simulink model "Intelligent_Microgrid_EMS"  (R2026b)
settings: Solver=FixedStepDiscrete  StopTime=24  FixedStep=1
undefined symbols (not defined in the file or in its folder): DiscIntNeverNeededParam
settings Model: Creator=Areeha  LastModifiedBy=Areeha

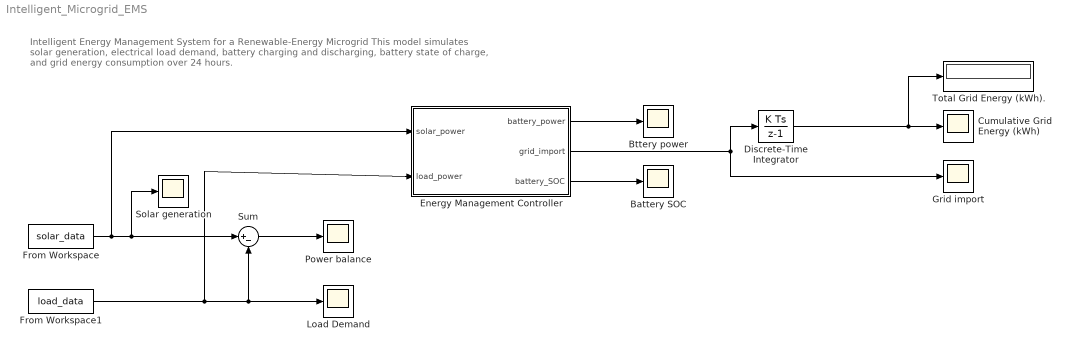
== system Intelligent_Microgrid_EMS ==
  note: Intelligent Energy Management System for a Renewable-Energy Microgrid This model simulates solar generation, electrical load demand, battery charging and discharging, battery state of charge, and grid energy consumption over 24 hours.
  Battery SOC : Scope
      settings: ActiveDisplayYMinimum=10.000000000000004  ActiveDisplayYMaximum=110  DataLoggingVariableName=ScopeData3
  Bttery power : Scope
      settings: ActiveDisplayYMinimum=-2.275  ActiveDisplayYMaximum=2.475
  Cumulative Grid Energy (kWh) : Scope
      settings: ActiveDisplayYMinimum=-2.2249999999999996  ActiveDisplayYMaximum=20.025000000000002  DataLoggingVariableName=ScopeData6
  Discrete-Time Integrator : DiscreteIntegrator  ICPrevOutput=DiscIntNeverNeededParam  ICPrevScaledInput=DiscIntNeverNeededParam
  Energy Management Controller : MATLAB Function  TreatAsAtomicUnit=on
  From Workspace : FromWorkspace  VariableName=solar_data
  From Workspace1 : FromWorkspace  VariableName=load_data
  Grid import : Scope
      settings: ActiveDisplayYMinimum=-0.37499999999999989  ActiveDisplayYMaximum=3.375  DataLoggingVariableName=ScopeData2
  Load Demand : Scope
      settings: ActiveDisplayYMinimum=0.40000000000000013  ActiveDisplayYMaximum=4.4  DataLoggingVariableName=ScopeData5
  Power balance : Scope
      settings: ActiveDisplayYMinimum=-4.725  ActiveDisplayYMaximum=2.525
  Solar generation : Scope
      settings: ActiveDisplayYMinimum=-0.62499999999999989  ActiveDisplayYMaximum=5.625  DataLoggingVariableName=ScopeData4
  Sum : Sum  Inputs=|+-
  Total Grid Energy (kWh). : Display
  wires:
  From Workspace/1 -> Energy Management Controller/1(solar_power), Solar generation/1, Sum/1
  From Workspace1/1 -> Load Demand/1, Sum/2, Energy Management Controller/2(load_power)
  Sum/1 -> Power balance/1
  Energy Management Controller/1(battery_power) -> Bttery power/1
  Energy Management Controller/2(grid_import) -> Grid import/1, Discrete-Time Integrator/1
  Energy Management Controller/3(battery_SOC) -> Battery SOC/1
  Discrete-Time Integrator/1 -> Total Grid Energy (kWh)./1, Cumulative Grid Energy (kWh)/1

== matlab function Intelligent_Microgrid_EMS/Energy Management Controller ==
  data: solar_power input; battery_power output; load_power input; grid_import output; battery_SOC output

function [battery_power, grid_import, battery_SOC] = fcn(solar_power, load_power)
% Intelligent Microgrid Energy Management Controller
% Battery power: negative = charging; positive = discharging
% SOC is the battery state of charge (%)

% Battery parameters
battery_capacity = 10;       % kWh
minimum_SOC = 20;            % %
maximum_SOC = 100;           % %
initial_SOC = 50;            % %
maximum_charge_power = 2;    % kW
maximum_discharge_power = 2; % kW
time_step = 1;               % hours
efficiency = 0.95;

% Persistent variable stores SOC between simulation steps
persistent SOC

if isempty(SOC)
    SOC = initial_SOC;
end

power_balance = solar_power - load_power;

% Determine battery action
if power_balance > 0
    % Charge only if the battery is not full
    if SOC < maximum_SOC
        battery_power = -min(power_balance, maximum_charge_power);
    else
        battery_power = 0;
    end

    grid_import = 0;

elseif power_balance < 0
    % Discharge only if SOC is above its minimum
    if SOC > minimum_SOC
        battery_power = min(-power_balance, maximum_discharge_power);
    else
        battery_power = 0;
    end

    grid_import = max(-power_balance - battery_power, 0);

else
    battery_power = 0;
    grid_import = 0;
end

% Update SOC
if battery_power < 0
    % Charging
    SOC = SOC + ((-battery_power) * efficiency * time_step ...
        / battery_capacity) * 100;

elseif battery_power > 0
    % Discharging
    SOC = SOC - ((battery_power / efficiency) * time_step ...
        / battery_capacity) * 100;
end

% Enforce SOC limits
SOC = min(max(SOC, minimum_SOC), maximum_SOC);

battery_SOC = SOC;
end
